simulink model "sem_harmonic_22a_mdl"  (R2022a)
settings: Solver=ode15s  StartTime=0.0  StopTime=5  RelTol=1e-3
settings Model: Creator=alinaakimkina
settings ModelReferenceCC: EnableRefExpFcnMdlSchedulingChecks=off
settings RTWCC: Description=Generic Real-Time Target

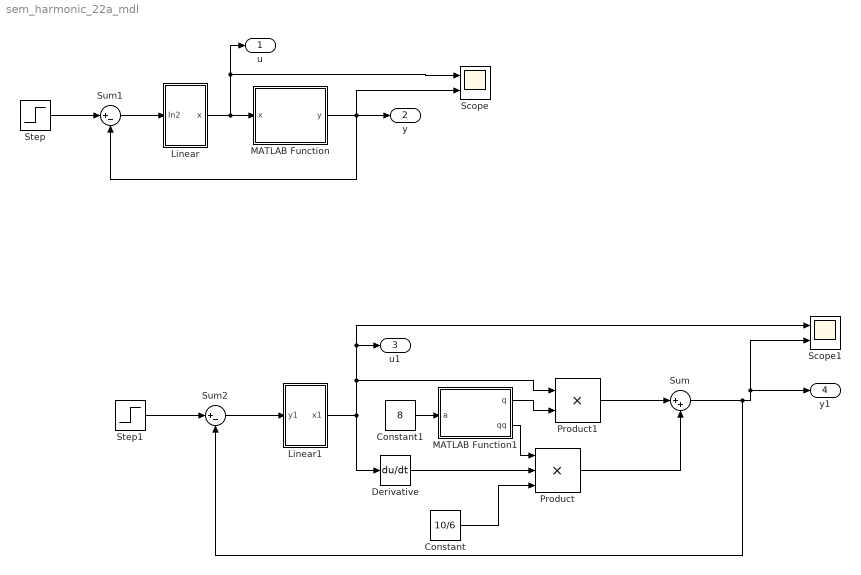
== system sem_harmonic_22a_mdl ==
  Constant : Constant  Value=10/6
  Constant1 : Constant  Value=8
  Derivative : Derivative
  Linear : Subsystem
  Linear1 : Subsystem
  MATLAB Function : MATLAB Function  TreatAsAtomicUnit=on
  MATLAB Function1 : MATLAB Function  TreatAsAtomicUnit=on
  Product : Product  Inputs=3
  Product1 : Product
  Scope : Scope  NumInputPorts=2
  Scope1 : Scope  NumInputPorts=2
  Step : Step  Time=0  After=0  SampleTime=0
  Step1 : Step  Time=0  After=0  SampleTime=0
  Sum : Sum  Inputs=|++
  Sum1 : Sum  Inputs=|+-
  Sum2 : Sum  Inputs=|+-
  u : Outport
  y : Outport  Port=2
  u1 : Outport  Port=3
  y1 : Outport  Port=4
  wires:
  MATLAB Function/1(y) -> y/1, Scope/2, Sum1/2
  Step/1 -> Sum1/1
  Sum1/1 -> Linear/1(In2)
  Linear/1(x) -> u/1, Scope/1, MATLAB Function/1(x)
  MATLAB Function1/2(qq) -> Product/1
  Constant/1 -> Product/3
  Derivative/1 -> Product/2
  Linear1/1(x1) -> Derivative/1, Product1/1, u1/1, Scope1/1
  Sum2/1 -> Linear1/1(y1)
  Step1/1 -> Sum2/1
  Constant1/1 -> MATLAB Function1/1(a)
  Product/1 -> Sum/2
  MATLAB Function1/1(q) -> Product1/2
  Product1/1 -> Sum/1
  Sum/1 -> Sum2/2, Scope1/2, y1/1

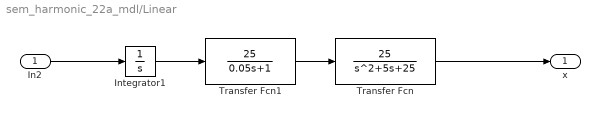
== system sem_harmonic_22a_mdl/Linear ==
  In2 : Inport
  Integrator1 : Integrator  InitialCondition=1
  Transfer Fcn : TransferFcn  Numerator=[25]  Denominator=[1 5 25]
  Transfer Fcn1 : TransferFcn  Numerator=[25]  Denominator=[0.05 1]
  x : Outport
  wires:
  Integrator1/1 -> Transfer Fcn1/1
  Transfer Fcn/1 -> x/1
  Transfer Fcn1/1 -> Transfer Fcn/1
  In2/1 -> Integrator1/1

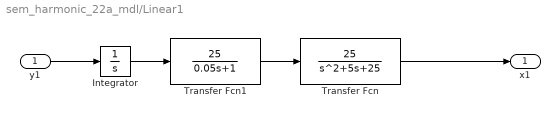
== system sem_harmonic_22a_mdl/Linear1 ==
  y1 : Inport
  Integrator : Integrator  InitialCondition=1
  Transfer Fcn : TransferFcn  Numerator=[25]  Denominator=[1 5 25]
  Transfer Fcn1 : TransferFcn  Numerator=[25]  Denominator=[0.05 1]
  x1 : Outport
  wires:
  y1/1 -> Integrator/1
  Transfer Fcn/1 -> x1/1
  Transfer Fcn1/1 -> Transfer Fcn/1
  Integrator/1 -> Transfer Fcn1/1

== matlab function sem_harmonic_22a_mdl/MATLAB Function1 ==
  data: a input; q output; qq output
function [q, qq]= fcn(a)
q = (4*1)/(pi*a)*sqrt(1 - 1/a^2);
qq = (4*1*1)/(pi*a^2);
% qq = (2/pi*a)*(-2*1*(1/a)+1*sin(15.5));
% q = (2*1/pi*a)*(2*sqrt(1-(1/a^2))-1-cos(15.5));
end

== matlab function sem_harmonic_22a_mdl/MATLAB Function ==
  data: y output; x input
function y = rele(x)
b = 1;
c = 1;
y = 0;
    if x >= b
        y = c;
    elseif x < b && x > 0
        y = -c;
    elseif x > -b && x <= 0
        y = c;
    elseif x < -b
        y = -c;
    end
end
